simulink model "commhdlQPSKTxRxLoopback"  (R2025b)
settings: Solver=FixedStepDiscrete  StartTime=0.0  StopTime=stopTime  RelTol=1e-3
PostLoadFcn:
  | hScopeConfig = get_param([gcs '/Receiver/QPSK Rx/Frequency and Time Synchronizer/Symbol Synchronizer/No HDL/QPSK Receiver Eye Diagram'],'ScopeConfiguration');
  | 
  | hScopeConfig.OpenAtSimulationStart = false;
  | hScopeConfig.Visible = false;
  | SamplesPerSymbol = 4;
  | %UpsamplesRx = 1;
  | clear hScopeConfig
InitFcn:
  | commhdlQPSKTxRxModelInit;
  | % Rate bridge: ADRV9002/Jupiter radio runs at 15.36 MHz = 2x the 7.68 MHz
  | % (4 samples/symbol @ Rsym=1.92 MHz) the QPSK Rx requires. The deployed
  | % Receiver must downsample the ADC stream by 2. UpsamplesRx=1 fed the QPSK
  | % Rx 8 sps (2x-upsampled) and broke symbol sync / the loopback bit check.
  | UpsamplesRx = 1;   %% T8 RATE FIX: rail 15.36e6 == ADC bus rate,
  | %% no ingress decimation (was 2 when the rail sat on the 7.68e6 rung)
  | UpsamplesTx = 1;
  | clear simTimingOffset;
StopFcn:
  | if exist('simTimingOffset','var')
  |   disp('Simulation completed');
  |   %QPSKTxRxVerification;
  | end
undefined symbols (not defined in the file or in its folder): Add, Config, fsym, randsrc, RandStream, Rsym, Shift
libraries: hdlsllib x141, simulink x43, dspsigops x34, dsphdlfiltering2 x6, dsphdlsigops2 x4, dsphdlmathfun2 x4, commdigbbndpm3 x4, dspmlti4 x2, commchan3 x1, commrflib2 x1, commcnvcod2 x1
(part 7 of 8)

== matlab function commhdlQPSKTxRxLoopback/TxRxComposite/Transmitter/Input Data/Message Generator/MATLAB Function ==
  data: enable input; reset input; out output; start output; stop output; valid output; count_out output; msg_count_out output
function [out, start, stop, valid, count_out, msg_count_out] = msggen(enable, reset)

persistent indexCount;
persistent toggle;
persistent msgCount;
persistent msgCountAll;
persistent msgCountBitIndex;

if isempty(indexCount) || isempty(toggle) || isempty(msgCount) || isempty(msgCountBitIndex) || isempty(msgCountAll)
    indexCount = uint32(0);
    msgCount = uint32(1);
    msgCountAll = uint32(1);
    msgCountBitIndex = uint8(0);
    toggle = false;
end

%% Constants -- FIXED pre-coded K=5 packet ROM (rom_words_770_f1536.txt, 24640 bits,
%% word w = bits[32w..32w+31] MSB-first). Stored as 770 x uint32 packed words
%% (a large inline logical literal crashes the Stateflow compiler),
%% unpacked into the 24640-element msgbits logical ROM and indexed with the
%% STOCK msgbits(indexCount+1) pattern. Replaces the stock 120-bit message ROM.
%% Content: K=5 [35 23] rate-1/2 coded info(12292)+tail(4) -> 24592 bits,
%% 1537x16 block-interleaved (perm r*16+c), + 48-bit PN9 filler. The K=5 Rx
%% deint(perm c*1537+r) + Viterbi(TB=25) recovers the 120-bit BIST message.
romWords = uint32([1204774986 2628405925 554197542 497400430 3820996551 1221748015 2714990298 259515120 3204786136 1111747194 4265078083 2294061781 4252484111 1721148643 1557893860 2008503539 2846627651 3001288225 3608790069 3556344180 2110069204 953332885 1538372371 3729622172 3587583480 2271786194 2977718194 1348372668 2426036822 1212264446 3479632192 3945694248 146715858 66061989 1158569579 2616330249 1320555108 3805748206 240428658 3122285248 1299730390 3039860570 771131690 2822406337 4290661082 2202099387 1549769405 2893845989 2600998515 1200035258 1094107672 1099071980 3265008536 2410273076 211921841 3201301283 3732450805 450863460 3808790566 2960537398 3321481865 2122952525 1387176159 1143071442 2099631177 2056641042 2863641865 1231021455 376307909 2197616876 2437410101 3473231534 1707820516 2804199802 4287800970 525245512 4287400560 941733719 2353727255 98958867 2441609524 1877563057 3458874722 4188353559 105620265 2074471427 1983048857 720775365 1107546864 4186768650 4288099257 1794542376 3585370352 3044414555 2973237059 438542858 663684233 4210999825 3687383987 2255322999 126746480 3874147988 3557246437 2327814052 2259727769 529243390 3139808402 1019349601 2913468750 3776145438 3218192218 1679393486 3688748042 901720909 839412932 92549236 4143869516 1934824460 1788212287 1942769059 1013575849 4110032482 563053040 1850769809 3240488323 2714138779 3171475398 2388251191 1287499602 2021425911 1663633101 2002380262 1487753104 2246178129 1703254886 492327426 2325492332 2800490288 3855795855 2775932910 529157251 1196838802 2389495825 2572500611 2575775365 1699514222 108536952 2750430041 4181752401 1819429509 2974747839 355458965 2012678107 2065033890 2844786194 3112234506 448673660 1484836811 2565291703 2094477854 3409179015 3327510003 3061116728 1944795825 2928127174 3552699018 2826263714 1931323920 2645996902 3881268263 725387150 4088705762 1959664038 612041663 3911000564 2257654739 3351079667 3084688792 3456682010 1882276373 3687344633 284287204 1736971757 3103109075 4280140713 2034865353 418309356 3396932588 1653019787 2489749539 3630574176 4241866407 260297666 2207592771 1611613421 2911869622 3858688321 2102485348 2606470610 1176244465 1972735515 1070738434 351822450 561779589 3717736920 1859230250 4190007144 3344666225 3718908926 1809913940 1552395775 170097309 3420266284 1291195965 414060454 3151636196 4181278958 69544123 1722966976 41363848 2052701966 2148240930 4210020045 1643657000 1434007316 2347774674 3570790404 2646965859 460251005 539614019 1888233478 1288955089 3958237818 1648780214 1688035146 855190402 4260566109 1992029421 3644403845 1457796463 707712161 2823206006 1846212180 1982008497 2947687159 3226916667 4197619858 4061717247 1762791550 51771752 1278696143 2864974893 770780492 3533740632 3702846591 458139812 1644550038 2378873953 131264765 424436432 3448581319 3977084430 2800008767 2727081006 1655892854 2436086872 119146047 665050641 3437208595 1599135822 2504069279 388650233 3639789145 3240350459 4054822260 2241026101 2315674586 3729684387 1673449533 4151924669 1548927388 340442120 133565182 4200412650 4014554963 2830808994 3551506689 1060106442 1252542399 3144191027 1035991056 4177333083 1741372263 3444104152 2835757074 2700282813 4011008101 425083707 644064140 3120038514 52663435 441667303 1895325662 1263931564 2569151693 4193445321 3378052811 855702763 3838759059 3308062449 1762745925 482832492 4223184315 2644262910 1282602893 3423923583 650582707 2333083778 3611966168 146704471 2253469441 2443167931 2065993115 2080912288 1573737723 3314798495 1753118653 452812869 3716937464 4067956266 3742845879 778453385 2954915383 3282312798 938302038 253881325 2795823423 2048676349 1594677050 2892897791 3727926439 3354101939 4198775546 1311370449 660520948 1353333928 154880548 2183869470 3725060759 2775971433 2575221904 2416034488 1657646592 3975407894 3052635703 1492153189 1557243130 1990465897 3308726660 439225568 85633354 4136453725 1495386754 1238548381 2298304656 2764377392 3649873585 2855253402 352344240 4094790042 969194247 4109734163 2337406488 2052196884 1091394433 803488059 1420380632 3128826663 3300317325 3947491526 301996578 2469890012 364654923 1170711462 2101109723 2136067173 274042398 806681041 2016703426 65809425 3192195138 3137859966 327888233 4194535610 3421255874 3294504871 2140344047 1986028453 3808044794 2446014534 3404471016 3822490226 104670575 1409213923 1771815875 1861397759 3161897377 600711989 2495113862 98524199 3813251024 2671722550 2817217516 3002574443 2519927130 3407407452 2312290502 407193247 4039266755 501354262 3932288117 2756321076 2418573729 2458706003 1768535580 1207610603 1938379566 1394731687 722817691 1156560878 3578824878 152882305 1969362243 1045935806 1919909200 2553299454 1691462377 384797729 342156685 4135847569 2752480027 572456332 1200746083 453259896 1173847343 2353570240 459967769 2229718858 234583034 3737354549 641363899 905708352 870591043 3816338511 4226902414 2944636663 2336637460 2639437974 4034472609 2625303238 405966835 434115564 2344572364 3290037663 892007983 1420432470 3298821096 4132420023 273983924 1532258286 953608378 830848693 338305776 248034844 246724321 2408799048 736838628 2806770526 1644065415 4176725552 2124475767 3595325100 2188919204 2600844190 1349260617 2465252426 681074018 3138380009 1254671038 2934970439 1755881642 2769505031 461276217 185413998 3689401219 1367446192 571090872 1964780208 3814307016 757034307 3302748047 762001668 3679735498 728484025 766308866 748968577 674652066 2692869255 2517922336 1176671792 439389165 275378995 2836149972 490199459 3418377363 2021597030 1122295240 3220148284 3587762966 2983976142 2996338941 1116580303 3675641017 4198486036 4137897679 685212839 2993855123 2423958832 2455239403 2542605922 3900485849 3144938974 3276808451 2606275657 1746710520 1838688044 2077093415 4219364598 4244533891 1670316944 1079359898 2000045550 1670044149 188287566 2387254478 4261053412 2934638187 169533072 186361277 1903326275 4188630055 256552686 2091365340 1887121706 2640438865 3842184106 2951323892 2513539091 2511150141 781332531 542618297 2808902628 2978110120 2333290371 4245887000 93692904 1794984085 2489138070 3630290001 1119726474 2949617493 2134020159 236835366 3830512295 2972725471 3770706533 164082753 2865844902 1963690776 547110901 68479344 2796641984 2157190697 2932488526 2565680122 199251104 2750385936 802045313 3487181851 3597940860 475550533 1731466611 617462254 1433761826 836633181 1254421314 4038005858 3758110602 1598484844 1764036035 1295413010 3612526779 3138044946 1487254459 2108728938 848239132 1884273911 806105759 2310209825 2793858610 142930553 1553760878 3765966331 1562125418 2195476893 98469432 12906494 771062714 2253495211 1508761233 1665010205 3343992922 648068057 4112097869 3902847612 1022478996 3591990475 1950414917 2290204022 3154386784 871299472 1308337656 3033065682 4037020892 901499362 293410562 2019718569 954362259 339324018 519334800 1419073632 3395549952 3113043604 1078022679 810475512 1680482793 3700335650 2071919666 3304054863 1221237577 3975557103 2288714635 1595764409 4272200962 1337052842 1448452549 1029713775 2675256063 2684707814 1138561228 3133255109 2040218036 2220298315 310391 3106542365 377013759 2931553628 3732706256 3361158608 39619392 1901289326 2461657569 391876191 4064810655 2713048210 2936763192 2804600942 2365800552 2185854409 2722164045 753728523 2696644393 3850641401 4080146876 1374584058 3196598824 3331963406 1038394409 3579841592 3165824404 1180665147 4001736500 1321078348 3862082772 1172264154 818506928 2212852913 399604020 57201615 103247012 3640764147 694436346 4272012647 316665873 82210424 3660906122 3449235625 3501281049 629142576 1125610876 426370477 1297644825 1906733320 1681235753 3340101163 3791793856 1591759449 2684862014 678672541 461395676 87629339 423207683 3845784129 529695163 756923300 1075034517 2811004745 854540833 2400148390 116007136 3496921158 749261405 3687467187 3133898680 295628066 1131078894 1959427393 885629835 1375667949 3684017968 1031834568 2286756503 2220869458 312242760 2857537372 99505339 1055291367 2596856259 1592613546 2990718201 1937257331 2787897945 4159425166 2898109988 1035418457 3161449681 1840239700 1902395198 433815854 594493721 2222399192 4293104410 1184159980 2612470674 2702705650 2972371074 1574626069 3945937279 1167261571 3742839305]);
msgbits = false(1,24640);
for w = 0:769
    wv = romWords(w+1);
    for bb = 0:31
        msgbits(w*32 + bb + 1) = bitget(wv, 32 - bb) ~= uint32(0);
    end
end
msgbitsLen = uint32(length(msgbits));

fullMessageLen = uint32(24640-1); %% Need the -1 to eat the feedback delay (stock hardcoded value in this model)

%% Logic
if enable && ~reset
    %% Set out data
    if indexCount < msgbitsLen %% Emit the fixed pre-coded packet bit (unpacked ROM)
        out = msgbits(indexCount + 1);
        msgCountBitIndex = uint8(0);
    else %% beyond the ROM (should not occur: msgbitsLen==dataBitsPerPacket)
        out = false;
        msgCountBitIndex = uint8(0);
    end

    %% Flags
    start = indexCount == uint32(0);
    stop = indexCount == fullMessageLen;
    valid = true;

    %% Counters
    if fullMessageLen == indexCount
        if msgCount >= 9
            msgCount = uint32(1);
        else
            msgCount = msgCount +  1;
            msgCountAll = msgCountAll + 1;
        end
    end
    if indexCount <= fullMessageLen
        indexCount = indexCount + 1;
    end

else %% Enable == false

    if reset
        indexCount = uint32(0);
        msgCountBitIndex = uint8(0);
        toggle = false;
    end
    out = false;
    start = false;
    stop = false;
    valid = false;
end

if isempty(indexCount)
    count_out = uint32(0);
else
    count_out = indexCount;
end

msg_count_out = msgCountAll;

== matlab function commhdlQPSKTxRxLoopback/Receiver/QPSK Rx/Frequency and Time Synchronizer/Preamble Detector/FIFO/Validate Input Push Pop/MATLAB Function ==
  data: rst input; count output; enb input; dir input; initVal parameter; countToVal parameter
function count = hdlCounter(rst,enb,dir,initVal,countToVal)
%#codegen

persistent countReg

if(isempty(countReg))
    countReg = fi(initVal,0,nextpow2(countToVal+1),0);
end

if(rst)
    countReg(:) = initVal;
elseif(enb)
    if(dir)
        if(countReg==countToVal)
            countReg(:) = initVal;
        else
            countReg(:) = countReg+1;
        end
    else
        if(countReg==initVal)
            countReg(:) = countToVal;
        else
            countReg(:) = countReg-1;
        end
    end
end

count = countReg;

end

== matlab function commhdlQPSKTxRxLoopback/Receiver/QPSK Rx/Frequency and Time Synchronizer/Preamble Detector/FIFO/Validate Input Push Pop/No HDL/MATLAB Function ==
  data: pushFullDiag input; popEmptyDiag input; pushFull input; popEmpty input
function pushPopDiagnostics(pushFullDiag, popEmptyDiag, pushFull, popEmpty)
%#codegen


if(pushFull)
    switch pushFullDiag
        case 2
            warning('Push signal applied on full FIFO');
        case 3
            error('Push signal applied on full FIFO');
        otherwise
    end
end

if(popEmpty)
    switch popEmptyDiag
        case 2
            warning('Pop signal applied on empty FIFO');
        case 3
            error('Pop signal applied on empty FIFO');
        otherwise
    end
end

end

== matlab function commhdlQPSKTxRxLoopback/TxRxComposite/Transmitter/QPSK Tx/Bit Packetizer/Data Bits FIFO/MATLAB Function1 ==
  data: wr input; full output; rd input; dataBitsPerPacket parameter
function full = fcn(wr,rd,dataBitsPerPacket)
%#codegen
     
    depth = dataBitsPerPacket*2 - 1;
    persistent count;
    if isempty(count)
        count = fi(0,0,nextpow2(depth),0,hdlfimath);
    end

    if wr
        count(:) = count + 1;
    end
    if rd
        count(:) = count - 1;
    end

    full = (count > depth);

end

== matlab function commhdlQPSKTxRxLoopback/Transmitter/QPSK Tx/Bit Packetizer/Data Bits FIFO/No HDL/MATLAB Function ==
  data: wr input; full output; rd input; ncount output; empty output; dataBitsPerPacket parameter
function [full,ncount,empty] = fcn(wr,rd,dataBitsPerPacket)
%#codegen
     
    depth = dataBitsPerPacket*2 - 1;
    persistent count;
    if isempty(count)
        count = fi(0,0,nextpow2(depth),0,hdlfimath);
    end

    empty = (count == 0);
    full = (count > depth);
    ncount = count;

    if wr
        count(:) = count + 1;
    end
    if rd
        count(:) = count - 1;
    end

end

== matlab function commhdlQPSKTxRxLoopback/TxRxComposite/Transmitter/QPSK Tx/Bit Packetizer/Data Bits FIFO/No HDL/MATLAB Function ==
  data: wr input; full output; rd input; ncount output; empty output; dataBitsPerPacket parameter
function [full,ncount,empty] = fcn(wr,rd,dataBitsPerPacket)
%#codegen
     
    depth = dataBitsPerPacket*2 - 1;
    persistent count;
    if isempty(count)
        count = fi(0,0,nextpow2(depth),0,hdlfimath);
    end

    empty = (count == 0);
    full = (count > depth);
    ncount = count;

    if wr
        count(:) = count + 1;
    end
    if rd
        count(:) = count - 1;
    end

end

== matlab function commhdlQPSKTxRxLoopback/TxRxComposite/Transmitter/QPSK Tx/Bit Packetizer/Data Bits FIFO/RAM Frame Status Indicator ==
  data: push input; out output; pop input; dataBitsPerPacket parameter
function out = fcn(push,pop,dataBitsPerPacket)

   persistent pushCount popCount frameCount;
   if isempty(pushCount)
       pushCount = fi(0,0,nextpow2(dataBitsPerPacket),0,hdlfimath);
       frameCount = fi(0,0,2,0,hdlfimath);
       popCount = fi(0,0,nextpow2(dataBitsPerPacket),0,hdlfimath);
   end
   
   if (pushCount == dataBitsPerPacket-1) && push
       frameCount(:) = frameCount + 1;
   end
   if (popCount == dataBitsPerPacket-1) && pop
       frameCount(:) = frameCount - 1;
   end

   if push
       if pushCount == dataBitsPerPacket - 1
           pushCount(:) = 0;
       else
           pushCount(:) = pushCount + 1;
       end
   end

   if pop 
       if popCount == dataBitsPerPacket - 1
           popCount(:) = 0;
       else
           popCount(:) = popCount + 1;
       end
   end

   out = frameCount;

end

== matlab function commhdlQPSKTxRxLoopback/TxRxComposite/Receiver/Capture Data Bits/MATLAB Function ==
  data: valid input; datain input; start input; stop input; count_out output; packets_out output; bit_errors_out output
function [count_out, packets_out, bit_errors_out] = msgdec(valid, datain, start, stop)

persistent count;
persistent msgbuffer;

persistent packetsReceived
persistent errors;

if isempty(count) || isempty(msgbuffer) || isempty(packetsReceived)
    count = uint32(0);
    msgbuffer = zeros(1,120+8)>0; % ADI Hello WorldX
    packetsReceived = uint32(0);
    errors = uint32(0);
end

% Mesg
strAscii = dec2bin('ADI Hello World',8);
msgarray = reshape(strAscii', [1, numel(strAscii)]);
msgbits = logical(msgarray - 48);

% msgLen = uint32(2240);

if valid
    if start
        count = uint32(1);
        packetsReceived = packetsReceived + 1;
    end

    if count <= (length(msgbuffer) - 8)
        msgbuffer(count) = datain;
        if datain ~= msgbits(count)
            errors = errors + 1;
        end

    elseif count == length(msgbuffer) + 1
        msgarray_dec = char('0' + msgbuffer);
        N = length(msgarray_dec) / 8;
        strAscii_dec = reshape(msgarray_dec , 8, N).';
        msg = char(bin2dec(strAscii_dec).');
        disp(msg);
    end
    
    if count <= length(msgbuffer) + 2
        count = count + 1;
    end
end

count_out = count;
packets_out = packetsReceived;
bit_errors_out = errors;

== matlab function commhdlQPSKTxRxLoopback/TxRxComposite/Receiver/QPSK Rx/Frequency and Time Synchronizer/Packet Controller/MATLAB Function ==
  data: valid input; syncPulse input; out output
function out = fcn(valid,syncPulse)
%#codegen

  persistent Reg;
  if isempty(Reg)
      Reg = false;
  end
  
  out = Reg;
  
  if Reg && valid
      Reg = false;
  end
  
  if syncPulse
      Reg = true;
  end
  
end

== matlab function commhdlQPSKTxRxLoopback/TxRxComposite/Receiver/QPSK Rx/Frequency and Time Synchronizer/Packet Controller/sample discard controller ==
  data: dataIn input; validIn input; dataOut output; startIn input; endIn input; startOut output; endOut output; validOut output
function [dataOut,startOut,endOut,validOut] = controller(dataIn,validIn,startIn,endIn)
%#codegen

   persistent active dataOutReg validOutReg startOutReg endOutReg;
   if isempty(active)
      active  = false;
      dataOutReg = cast(0,'like',dataIn);
      validOutReg = false;
      startOutReg = false;
      endOutReg = false;
   end
   
   dataOut = dataOutReg;
   validOut = validOutReg;
   startOut = startOutReg;
   endOut = endOutReg;
   
   startOutReg = startIn;
   endOutReg = endIn;
   
   if startIn
       active = true;
   end
   
   if active
       dataOutReg(:) = dataIn;
       validOutReg = validIn;
   else
       dataOutReg(:) = 0;
       validOutReg = false;
   end
   
   if endIn
       if active 
           endOutReg = true;
       else
           endOutReg = false;
       end
       active = false;
   end
end

== matlab function commhdlQPSKTxRxLoopback/TxRxComposite/Receiver/QPSK Rx/Frequency and Time Synchronizer/Preamble Detector/Correlator/ThresholdLimiter ==
  settings: fimath=hdlfimath
  data: x input; y output
function y = applyLowerLimit(x)
    % Apply a lower limit to the threshold.
    %#codegen
    
    % Threshold is computed by summing across 63 samples.
    % Set lower limit to be equivalent of all 63 samples
    % having their LSB set to 1 and all others set to 0. 
    lowerLimit = cast(0.01, 'like', x);
    
    if x < lowerLimit
        y = lowerLimit;
    else
        y = x;
    end
end

== matlab function commhdlQPSKTxRxLoopback/TxRxComposite/Receiver/QPSK Rx/Frequency and Time Synchronizer/Preamble Detector/FIFO/Validate Input Push Pop/MATLAB Function ==
  data: rst input; count output; enb input; dir input; initVal parameter; countToVal parameter
function count = hdlCounter(rst,enb,dir,initVal,countToVal)
%#codegen

persistent countReg

if(isempty(countReg))
    countReg = fi(initVal,0,nextpow2(countToVal+1),0);
end

if(rst)
    countReg(:) = initVal;
elseif(enb)
    if(dir)
        if(countReg==countToVal)
            countReg(:) = initVal;
        else
            countReg(:) = countReg+1;
        end
    else
        if(countReg==initVal)
            countReg(:) = countToVal;
        else
            countReg(:) = countReg-1;
        end
    end
end

count = countReg;

end

== matlab function commhdlQPSKTxRxLoopback/TxRxComposite/Receiver/QPSK Rx/Frequency and Time Synchronizer/Preamble Detector/FIFO/Validate Input Push Pop/No HDL/MATLAB Function ==
  data: pushFullDiag input; popEmptyDiag input; pushFull input; popEmpty input
function pushPopDiagnostics(pushFullDiag, popEmptyDiag, pushFull, popEmpty)
%#codegen


if(pushFull)
    switch pushFullDiag
        case 2
            warning('Push signal applied on full FIFO');
        case 3
            error('Push signal applied on full FIFO');
        otherwise
    end
end

if(popEmpty)
    switch popEmptyDiag
        case 2
            warning('Pop signal applied on empty FIFO');
        case 3
            error('Pop signal applied on empty FIFO');
        otherwise
    end
end

end

== matlab function commhdlQPSKTxRxLoopback/Receiver/QPSK Rx/Frequency and Time Synchronizer/Packet Controller/MATLAB Function ==
  data: valid input; syncPulse input; out output
function out = fcn(valid,syncPulse)
%#codegen

  persistent Reg;
  if isempty(Reg)
      Reg = false;
  end
  
  out = Reg;
  
  if Reg && valid
      Reg = false;
  end
  
  if syncPulse
      Reg = true;
  end
  
end

== matlab function commhdlQPSKTxRxLoopback/TxRxComposite/Receiver/QPSK Rx/Frequency and Time Synchronizer/Symbol Synchronizer/Interpolation Control ==
  data: mu output; Delta input; Underflow output
function [mu,Underflow] = Interpolation_ctrl(Delta)
% Implementation of modulo-1 counter for interpolation control listed in
% Figure 8.4.19 of "Digital Communications - A Discrete-Time Approach"
% by Michael Rice. See design details in Chapter 8.4.3 of the same book.
% 
% Input:
%   Delta - Loop filter output. If loop is in lock, delta would be small
% Output:
%   Underflow - Indicator of counter underflow. This is the strobe signal
%               for downstream processing
%   mu - Difference between actual sampling instant and the optimal instant,
%        between zero and one
%#codegen

% countReg - Counter value delayed by 1 sample
% muReg - The estimated timing error normalized by half QPSK symbols

   mask = fi(1-2^(-10),1,11,10);
   
   persistent countReg underflowReg muReg;
   if isempty(countReg)
       countReg  = fi(0,1,11,10);
       muReg = fi(0,1,11,10);
       underflowReg = false;
   end
   
   
   Underflow = underflowReg;
   mu = muReg;   
   
   
      % T8.4 anti-wedge clamp: if Delta <= -0.125 the decrementing counter
   % never underflows (strobes stop FOREVER -- Class-4 wedge / Class-1
   % episode mechanism; see tb_timing_wedge.v). Bound Delta so the
   % counter always decrements by >= 1 LSB.
   wlim = fi(255/1024,1,11,10);
   if Delta > wlim
       Delta = wlim;
   elseif Delta < -wlim
       Delta = fi(-255/1024,1,11,10);
   end
   counter = bitand(mask,countReg)-Delta-fi(0.25,1,11,10); % decrementing counter
   
   % if countReg is a nonnegative number,
   % then mod(countReg,1) equals the fractional part of countReg
   if counter < 0
       underflowReg = true;
       muReg = bitshift(bitand(mask,countReg),2);
       countReg = fi(counter+1,1,11,10);% create underflow to counter
   else
       underflowReg = false;
       countReg = fi(counter,1,11,10);
   end
   


end

== matlab function commhdlQPSKTxRxLoopback/TxRxComposite/Receiver/QPSK Rx/Frequency and Time Synchronizer/Symbol Synchronizer/Rate Handle/FIFO/Validate Input Push Pop/MATLAB Function ==
  data: rst input; count output; enb input; dir input; initVal parameter; countToVal parameter
function count = hdlCounter(rst,enb,dir,initVal,countToVal)
%#codegen

persistent countReg

if(isempty(countReg))
    countReg = fi(initVal,0,nextpow2(countToVal+1),0);
end

if(rst)
    countReg(:) = initVal;
elseif(enb)
    if(dir)
        if(countReg==countToVal)
            countReg(:) = initVal;
        else
            countReg(:) = countReg+1;
        end
    else
        if(countReg==initVal)
            countReg(:) = countToVal;
        else
            countReg(:) = countReg-1;
        end
    end
end

count = countReg;

end

== matlab function commhdlQPSKTxRxLoopback/TxRxComposite/Receiver/QPSK Rx/Frequency and Time Synchronizer/Symbol Synchronizer/Rate Handle/FIFO/Validate Input Push Pop/No HDL/MATLAB Function ==
  data: pushFullDiag input; popEmptyDiag input; pushFull input; popEmpty input
function pushPopDiagnostics(pushFullDiag, popEmptyDiag, pushFull, popEmpty)
%#codegen


if(pushFull)
    switch pushFullDiag
        case 2
            warning('Push signal applied on full FIFO');
        case 3
            error('Push signal applied on full FIFO');
        otherwise
    end
end

if(popEmpty)
    switch popEmptyDiag
        case 2
            warning('Pop signal applied on empty FIFO');
        case 3
            error('Pop signal applied on empty FIFO');
        otherwise
    end
end

end

== matlab function commhdlQPSKTxRxLoopback/TxRxComposite/Receiver/QPSK Rx/FEC Decoder Wrapper/RxDeint ==
  data: dataIn input; codedPair output; startIn input; endIn input; validIn input; vitReset output; deintValid output; frameStart output; frameEnd output
function [codedPair, vitReset, deintValid, frameStart, frameEnd] = fecRxDeint(dataIn, startIn, endIn, validIn)
%#codegen
persistent ramA ramB rdBank wptr pcnt hold0 hold1 rdGate rcol rrow;
CODED=uint16(24592); COLS=uint16(16); ROWS=uint16(1537);
NPAIR=uint16(12296);
if isempty(ramA), ramA=fi(zeros(1,24592),0,1,0); ramB=fi(zeros(1,24592),0,1,0); rdBank=false; wptr=uint16(0); pcnt=uint16(0); hold0=fi(0,0,1,0); hold1=fi(0,0,1,0); rdGate=false; rcol=uint16(0); rrow=uint16(0); end
rb=rdBank; w=wptr; pc=pcnt; g=rdGate; h0=hold0; h1=hold1; cc=rcol; rr=rrow;
pair0=h0; pair1=h1;
vitReset=false; deintValid=false; frameStart=false; frameEnd=false;
wrPos=uint16(65535); wrBit=fi(0,0,1,0); wrBankA=false; doWr=false;
if validIn
  if startIn, w=uint16(0); pc=uint16(0); rb=~rb; g=true; cc=uint16(0); rr=uint16(0); end % rdGate=TRUE: frame pair0 read COINCIDES with frameStart (RxAlign arms on that beat); read-counters reset in lockstep with pc
  % ---- READ side first (opposite bank; RXROOT E8 isolated reads: 1 pair per 2 validIn beats) ----
  if g && (pc < NPAIR)
    % divisionless read address: cc (even col) / rr (row) are incremental counters.
    % rc0=2*pc is even so rc1=rc0+1 keeps the same row -> perm1 = perm0 + ROWS (one add).
    perm0 = cc*ROWS + rr;
    perm1 = perm0 + ROWS;
    b0v = fi(0,0,1,0); b1v = fi(0,0,1,0);
    if perm0 < CODED
      if rb, b0v = ramB(double(perm0)+1); else b0v = ramA(double(perm0)+1); end
    end
    if perm1 < CODED
      if rb, b1v = ramB(double(perm1)+1); else b1v = ramA(double(perm1)+1); end
    end
    pair0 = b0v; pair1 = b1v; h0 = b0v; h1 = b1v;
    deintValid = true;
    if pc == uint16(0), vitReset = true; end
    pc = pc + 1;
    cc = cc + uint16(2);
    if cc == COLS, cc = uint16(0); rr = rr + uint16(1); end
  end
  % ---- WRITE side after all reads ----
  if w < CODED
    wrPos = w; wrBit = fi(dataIn,0,1,0); wrBankA = rb; doWr = true;
    w = w + 1;
  end
  g = ~g;
  frameStart=startIn; frameEnd=endIn;
end
codedPair = fi([pair0; pair1], 0, 1, 0);
% ---- persist state last ----
if doWr
  if wrBankA, ramA(double(wrPos)+1)=wrBit; else ramB(double(wrPos)+1)=wrBit; end
end
rdBank=rb; wptr=w; pcnt=pc; rdGate=g; hold0=h0; hold1=h1; rcol=cc; rrow=rr;

== matlab function commhdlQPSKTxRxLoopback/TxRxComposite/Receiver/QPSK Rx/FEC Decoder Wrapper/RxAlign ==
  data: decBit input; dataOut output; deintValid input; frameStart input; frameEnd input; skipCount input; startOut output; endOut output; validOut output
function [dataOut, startOut, endOut, validOut] = fecRxAlign(decBit, deintValid, frameStart, frameEnd, skipCount)
%#codegen
persistent oc started skip;
INFO=uint16(12292);
if isempty(oc), oc=uint16(0); started=false; skip=uint16(0); end
o=oc; st=started; sk=skip;
dataOut=false; startOut=false; endOut=false; validOut=false;
sc = uint16(skipCount);
if sc > INFO, sc = INFO; end
if deintValid
  if frameStart, o=uint16(0); st=true; sk=sc+uint16(41); end % +41 = gated-Viterbi latency in deintValid beats incl. VitGate hold reg (RXROOT E8)
  if st
    if sk > uint16(0)
      sk = sk - uint16(1);
    elseif o < INFO
      dataOut = decBit;
      startOut = (o==uint16(0));
      endOut   = (o==(INFO-1));
      validOut = true;
      o = o + uint16(1);
    end
  end
end
oc=o; started=st; skip=sk;

== matlab function commhdlQPSKTxRxLoopback/TxRxComposite/Receiver/QPSK Rx/FEC Decoder Wrapper/FecCounters ==
  data: e1 input; c1 output; e2 input; e3 input; e4 input; e5 input; e6 input; c2 output; c3 output; c4 output; c5 output; c6 output
function [c1, c2, c3, c4, c5, c6] = fecCounters(e1, e2, e3, e4, e5, e6)
%#codegen
% Free-running FEC-Rx datapath event counters (reset by modem soft-reset 0x000).
persistent k1 k2 k3 k4 k5 k6;
if isempty(k1)
  k1=uint32(0); k2=uint32(0); k3=uint32(0); k4=uint32(0); k5=uint32(0); k6=uint32(0);
end
MAX=uint32(4294967295);
n1=k1; n2=k2; n3=k3; n4=k4; n5=k5; n6=k6;
if e1 && n1<MAX, n1=n1+uint32(1); end
if e2 && n2<MAX, n2=n2+uint32(1); end
if e3 && n3<MAX, n3=n3+uint32(1); end
if e4 && n4<MAX, n4=n4+uint32(1); end
if e5 && n5<MAX, n5=n5+uint32(1); end
if e6 && n6<MAX, n6=n6+uint32(1); end
c1=n1; c2=n2; c3=n3; c4=n4; c5=n5; c6=n6;
k1=n1; k2=n2; k3=n3; k4=n4; k5=n5; k6=n6;

== matlab function commhdlQPSKTxRxLoopback/Receiver/QPSK Rx/Frequency and Time Synchronizer/Symbol Synchronizer/Rate Handle/FIFO/Validate Input Push Pop/MATLAB Function ==
  data: rst input; count output; enb input; dir input; initVal parameter; countToVal parameter
function count = hdlCounter(rst,enb,dir,initVal,countToVal)
%#codegen

persistent countReg

if(isempty(countReg))
    countReg = fi(initVal,0,nextpow2(countToVal+1),0);
end

if(rst)
    countReg(:) = initVal;
elseif(enb)
    if(dir)
        if(countReg==countToVal)
            countReg(:) = initVal;
        else
            countReg(:) = countReg+1;
        end
    else
        if(countReg==initVal)
            countReg(:) = countToVal;
        else
            countReg(:) = countReg-1;
        end
    end
end

count = countReg;

end

== matlab function commhdlQPSKTxRxLoopback/TxRxComposite/Receiver/QPSK Rx/FEC Decoder Wrapper/FecCapture ==
  data: bitsIn input; capIn output; validIn input; startIn input; codedPair input; deintValid input; decBit input; skipCount input; outValid input; capDeint output; capOut output
function [capIn, capDeint, capOut] = fecCapture(bitsIn, validIn, startIn, codedPair, deintValid, decBit, skipCount, outValid)
%#codegen
persistent rIn rDe rOu nIn nDe nOu armIn skp;
if isempty(rIn)
  rIn=uint32(0); rDe=uint32(0); rOu=uint32(0);
  nIn=uint16(0); nDe=uint16(0); nOu=uint16(0); armIn=false; skp=uint16(0);
end
% sync-semantics compliant (RXROOT E11c): locals, persist last.
a=rIn; b=rDe; c=rOu; xIn=nIn; xDe=nDe; xOu=nOu; arm=armIn; sk=skp; %#ok<NASGU>
% --- CAP_IN: first 32 coded-in bits, armed at startIn, gated by validIn ---
if validIn
  if startIn, xIn=uint16(0); a=uint32(0); arm=true; end
  if arm && xIn < uint16(32)
    if bitsIn, a = bitor(a, bitshift(uint32(1), double(xIn))); end
    xIn = xIn + uint16(1);
  end
end
% --- CAP_DEINT: first 32 deint-output coded bits (2 per pair), gated by deintValid ---
if startIn, xDe=uint16(0); b=uint32(0); end
if deintValid && xDe < uint16(32)
  b0 = codedPair(1) ~= 0; b1 = codedPair(2) ~= 0;
  if b0, b = bitor(b, bitshift(uint32(1), double(xDe))); end
  xDe = xDe + uint16(1);
  if xDe < uint16(32)
    if b1, b = bitor(b, bitshift(uint32(1), double(xDe))); end
    xDe = xDe + uint16(1);
  end
end
% --- CAP_OUT (RXROOT E8): first 32 bits of the WRAPPER OUTPUT stream ---
% i6 = RxAlign dataOut gated by i8 = RxAlign validOut: exactly the bits the
% BIST compares, alignment-independent. Golden expectation 0x04922282.
sc = uint16(skipCount); sk = uint16(0); %#ok<NASGU>
if startIn, xOu=uint16(0); c=uint32(0); end
if outValid && xOu < uint16(32)
  if decBit, c = bitor(c, bitshift(uint32(1), double(xOu))); end
  xOu = xOu + uint16(1);
end
capIn = a; capDeint = b; capOut = c;
rIn=a; rDe=b; rOu=c; nIn=xIn; nDe=xDe; nOu=xOu; armIn=arm; skp=sk;

== matlab function commhdlQPSKTxRxLoopback/TxRxComposite/Receiver/QPSK Rx/FecCaptureCadence ==
  data: startIn input; capCad output; validIn input
function capCad = fecCaptureCadence(startIn, validIn)
%#codegen
persistent sCnt gap snv vrun seenStart sawValid measuring;
if isempty(sCnt)
  sCnt=uint8(0); gap=uint8(0); snv=uint8(0); vrun=uint8(0);
  seenStart=false; sawValid=false; measuring=false;
end
% sync-semantics compliant (RXROOT E11c): locals, persist last.
sC=sCnt; gp=gap; sv=snv; vr=vrun; seen=seenStart; saw=sawValid; mea=measuring;
if startIn
  if sC < uint8(255), sC = sC + uint8(1); end
  if ~validIn && sv < uint8(255), sv = sv + uint8(1); end
  if ~seen
    seen = true; mea = true; gp = uint8(0); saw=false; vr=uint8(0);
  end
end
if mea && ~saw
  if validIn
    saw = true;
  elseif gp < uint8(255)
    gp = gp + uint8(1);
  end
end
if seen && validIn && vr < uint8(255)
  vr = vr + uint8(1);
end
capCad = bitor(bitor(uint32(sC), bitshift(uint32(gp),8)), bitor(bitshift(uint32(sv),16), bitshift(uint32(vr),24)));
sCnt=sC; gap=gp; snv=sv; vrun=vr; seenStart=seen; sawValid=saw; measuring=mea;

== matlab function commhdlQPSKTxRxLoopback/TxRxComposite/Receiver/QPSK Rx/RstCsCounter ==
  data: e input; c output
function c = rstCsCount(e)
%#codegen
% Count RISING EDGES of the CFO-step-detector carrier-sync reset (AXI 0x150).
% Saturating; reset by the modem soft-reset 0x000 via the persistent init.
persistent prev cnt;
if isempty(prev), prev = false; cnt = uint32(0); end
n = cnt;
if e && ~prev && n < uint32(4294967295)
    n = n + uint32(1);
end
c = n;
cnt = n;
prev = logical(e);

== matlab function commhdlQPSKTxRxLoopback/TxRxComposite/Transmitter/Input Data/ByteBitShifter ==
  data: enable input; bit output; reset input; start input; extWord input; extWordAvail input; extWordFirst input; popToggle output
function [bit, popToggle] = byteBitShifterBlk(enable, reset, start, extWord, extWordAvail, extWordFirst)
% Block wrapper around qpskByteBitShifterStrict (the unit-tested single source
% of truth). Persistent state only; the effective enable matches the
% Message Generator chart's active condition (enable && ~reset) so the
% shifter emits bits on exactly the generator's bit steps. pop is
% exported as a toggle (one flip per word latch OR discard) to survive
% the slow->fast rate crossing; upstream edge-detects it into a pulse.
persistent state tog
if isempty(state)
    state = qpskByteBitShifterStrict();
    tog = false;
end
en = logical(enable) && ~logical(reset);
[bit, pop, state] = qpskByteBitShifterStrict(state, en, logical(start), ...
    uint64(extWord), logical(extWordAvail), logical(extWordFirst));
if pop
    tog = ~tog;
end
popToggle = tog;

== matlab function commhdlQPSKTxRxLoopback/TxRxComposite/Transmitter/Input Data/FEC Tx Encoder K5/TxGateK5 ==
  data: bitIn input; infoBit output; enable input; reset input; start input; encReset output; infoValid output; beatIdx output; frameValid output; frameStart output
function [infoBit, encReset, infoValid, beatIdx, frameValid, frameStart] = fecTxGateK5(bitIn, enable, reset, start)
%#codegen
% sync-semantics (RXROOT E11c): locals in, outputs from locals, persist last.
persistent beat armed;
INFO=uint16(12292); NIN=uint16(12296); PAYLOAD=uint16(24640);
if isempty(beat), beat=uint16(0); armed=false; end
b=beat; a=armed;
infoBit=false; encReset=false; infoValid=false; beatIdx=uint16(0);
frameValid=false; frameStart=false;
en = logical(enable) && ~logical(reset);
if en
  if start, b=uint16(0); a=true; encReset=true; end
  if a
    if b < INFO
      infoBit = logical(bitIn); infoValid = true;
    elseif b < NIN
      infoBit = false;          infoValid = true;   % K-1 zero tail flush
    end
    beatIdx = b; frameValid = true; frameStart = (b==uint16(0));
    if b < PAYLOAD-uint16(1), b=b+uint16(1); else, b=uint16(0); end
  end
end
beat=b; armed=a;

== matlab function commhdlQPSKTxRxLoopback/TxRxComposite/Transmitter/Input Data/FEC Tx Encoder K5/ConvEncK5 ==
  data: infoBit input; codedPair output; encReset input; infoValid input
function codedPair = fecConvEncK5(infoBit, encReset, infoValid)
%#codegen
persistent sr;
if isempty(sr), sr = false(1,4); end
srUse = sr;
if encReset, srUse = false(1,4); end   % reset-then-advance (zero frame state)
in = logical(infoBit);
s0=in; s1=srUse(1); s2=srUse(2); s3=srUse(3); s4=srUse(4);
g0 = xor(s0, xor(s1, xor(s2, s4)));   % poly 35 oct = 11101
g1 = xor(s0, xor(s3, s4));            % poly 23 oct = 10011
codedPair = [g0; g1];
% state update: advance ONLY on infoValid, else HOLD (anti-zero-stuff gate)
if infoValid
  sr = [in, srUse(1:3)];
else
  sr = srUse;
end

== matlab function commhdlQPSKTxRxLoopback/TxRxComposite/Transmitter/Input Data/FEC Tx Encoder K5/TxInterleaveK5 ==
  data: codedPair input; dataOut output; infoValid input; beatIdx input; frameValid input; frameStart input
function dataOut = fecTxInterleaveK5(codedPair, infoValid, beatIdx, frameValid, frameStart)
%#codegen
persistent ramA ramB rdBank wptr rrow rcol;
CODED=uint16(24592); COLS=uint16(16); ROWS=uint16(1537);
FILL = logical([1 1 1 1 1 1 1 1 1 0 0 0 0 0 1 1 1 1 0 1 1 1 1 1 0 0 0 1 0 1 1 1 0 0 1 1 0 0 1 0 0 0 0 0 1 0 0 1]);   % 64-bit PN9 filler (T8 fix 6bcaa62)
if isempty(ramA), ramA=fi(zeros(1,24592),0,1,0); ramB=fi(zeros(1,24592),0,1,0); rdBank=false; wptr=uint16(0); rrow=uint16(0); rcol=uint16(0); end
rb=rdBank; w=wptr; rr=rrow; cc=rcol;
dataOut=false;
wr0=uint16(0); wr1=uint16(0); v0=fi(0,0,1,0); v1=fi(0,0,1,0); doW0=false; doW1=false;
if frameValid
  if frameStart, w=uint16(0); rb=~rb; end
  % ---- READ side (previous frame, opposite bank), legacy perm r*COLS+c ----
  % divisionless read address: rr (row 0..ROWS-1) / cc (col 0..COLS-1) are
  % incremental counters, reset on beatIdx==0, advancing +1 row with col carry
  % per in-range beat -- replaces the old per-beat divide-by-ROWS. No divide.
  if beatIdx < CODED
    % precondition: bit-exactness requires a contiguous beatIdx hitting 0 once per
    % frame to re-seed the row/col counters (the old stateless per-beat address
    % arithmetic derived the address from beatIdx alone and needed no such reset).
    if beatIdx == 0, rr = uint16(0); cc = uint16(0); end
    perm = rr*COLS + cc;
    if perm < CODED
      if rb, dataOut = logical(ramB(double(perm)+1)); else, dataOut = logical(ramA(double(perm)+1)); end
    end
    rr = rr + uint16(1);
    if rr == ROWS, rr = uint16(0); cc = cc + uint16(1); end
  else
    dataOut = FILL(double(beatIdx-CODED)+1);   % PN9 filler, beats CODED..2239
  end
  % ---- WRITE side: two coded bits per encoder-advance beat ----
  if infoValid
    if w < CODED, wr0=w; v0=fi(double(codedPair(1)~=0),0,1,0); doW0=true; w=w+uint16(1); end
    if w < CODED, wr1=w; v1=fi(double(codedPair(2)~=0),0,1,0); doW1=true; w=w+uint16(1); end
  end
end
% ---- persist state last (write bank = opposite of read bank) ----
if doW0
  if rb, ramA(double(wr0)+1)=v0; else, ramB(double(wr0)+1)=v0; end
end
if doW1
  if rb, ramA(double(wr1)+1)=v1; else, ramB(double(wr1)+1)=v1; end
end
rdBank=rb; wptr=w; rrow=rr; rcol=cc;

== matlab function commhdlQPSKTxRxLoopback/TxRxComposite/ByteWordBuffer ==
  data: dataIn input; word output; validIn input; popReq input; firstIn input; avail output; readyNext output; wordFirst output
function [word, avail, readyNext, wordFirst] = byteWordBufferBlk(dataIn, validIn, popReq, firstIn)
% Block wrapper around qpskByteWordBufferSkid (unit-tested single source of
% truth); persistent state only. readyNext = the post-update registered
% ready; an external Delay (IC=1) turns it back into the AXIS tready.
% firstIn/wordFirst carry the in-band first-word marker alongside data.
persistent state
if isempty(state)
    state = qpskByteWordBufferSkid();
end
[word, avail, ~, wordFirst, state] = qpskByteWordBufferSkid(state, uint64(dataIn), ...
    logical(validIn), logical(popReq), logical(firstIn));
readyNext = state.readyReg;

== matlab function commhdlQPSKTxRxLoopback/TxRxComposite/ByteSerializer ==
  data: bitIn input; word output; bitValid input; start input; ready input; wordTog output; wordLast output; wordFirst output
function [word, wordTog, wordLast, wordFirst] = byteSerializerBlk(bitIn, bitValid, start, ready)
% Block wrapper around qpskByteSerializer (unit-tested single source of
% truth); persistent state only. word/wordLast are HELD stable between
% emissions; wordTog flips once per emitted word so the slow->fast rate
% crossing cannot drop or repeat it -- the 30.72M BeatGate edge-detects
% it into exactly one accepted AXIS beat. Dropped words (ready low at
% completion) do not toggle: drop means NO beat, never a stall.
% K5 kit: 191 words/frame = the first 64*191 of
% the 1084 decoded info bits; the trailing 60 are dropped by start-reset.
persistent state tog heldWord heldLast heldFirst firstNext
if isempty(state)
    state = qpskByteSerializer();
    tog = false; heldWord = uint64(0); heldLast = false;
    heldFirst = true; firstNext = true;
end
% presentation is decoupled from acceptance (ADI S2MM source style):
% the offered beat must refresh on EVERY completed word or the DMA's
% SYNC_TRANSFER_START gate can wait forever on a frozen user flag /
% accept a stale word. ready at the pin only decides acceptance, so
% the core serializer runs with ready=true and unaccepted beats are
% simply superseded.
[w, wv, wl, ~, state] = qpskByteSerializer(state, logical(bitIn), ...
    logical(bitValid), logical(start), true, uint16(191));
if wv
    heldWord = w; heldLast = logical(wl); tog = ~tog;
    heldFirst = firstNext; firstNext = logical(wl);
end
word = heldWord; wordTog = tog; wordLast = heldLast; wordFirst = heldFirst;

== matlab function commhdlQPSKTxRxLoopback/TxRxComposite/ByteRxFifo ==
  data: word input uint64; outWord output uint64; tog input boolean; wLast input boolean; wFirst input boolean; ready input boolean; valid output boolean; outLast output boolean; outFirst output boolean; ovf output uint32
function [outWord, valid, outLast, outFirst, ovf] = byteRxFifo(word, tog, wLast, wFirst, ready)
%#codegen
% 64-deep elastic FIFO: enqueue on serializer toggle edge, dequeue on
% accepted AXIS beat. Drop-newest + count on full (stall > ~19 ms).
% f1536 SOF-prime guard (TXMUX 2026-07-25): valid is presented only after
% ready has been continuously high for 6 cycles, so the axi_dmac S2MM
% per-descriptor SOF prime (5-cycle latency, replicates a HELD beat x5 =
% the W0x5 dup) never sees a held beat during its prime window.
persistent mem memFl wr rd prev ovfCnt rdyRun
if isempty(wr)
    mem = zeros(64,1,'uint64'); memFl = zeros(64,1,'uint8');
    wr = uint16(0); rd = uint16(0); prev = false; ovfCnt = uint32(0);
    rdyRun = uint8(0);
end
if logical(tog) ~= prev
    nxt = uint16(mod(uint32(wr) + 1, 64));
    if nxt == rd
        rd = uint16(mod(uint32(rd) + 1, 64));
        ovfCnt = ovfCnt + uint32(1);
    end
    mem(uint32(wr)+1)   = uint64(word);
    memFl(uint32(wr)+1) = uint8(wLast) + uint8(2)*uint8(wFirst);
    wr = nxt;
end
prev = logical(tog);
valid = (wr ~= rd) && (rdyRun >= uint8(6));
outWord  = mem(uint32(rd)+1);
fl = memFl(uint32(rd)+1);
outLast  = bitand(fl, uint8(1)) ~= uint8(0);
outFirst = bitand(fl, uint8(2)) ~= uint8(0);
if valid && logical(ready)
    rd = uint16(mod(uint32(rd) + 1, 64));
end
if logical(ready)
    if rdyRun < uint8(255), rdyRun = rdyRun + uint8(1); end
else
    rdyRun = uint8(0);
end
ovf = ovfCnt;

== matlab function commhdlQPSKTxRxLoopback/Transmitter/QPSK Tx/Bit Packetizer/Data Bits FIFO/MATLAB Function1 ==
  data: wr input; full output; rd input; dataBitsPerPacket parameter
function full = fcn(wr,rd,dataBitsPerPacket)
%#codegen
     
    depth = dataBitsPerPacket*2 - 1;
    persistent count;
    if isempty(count)
        count = fi(0,0,nextpow2(depth),0,hdlfimath);
    end

    if wr
        count(:) = count + 1;
    end
    if rd
        count(:) = count - 1;
    end

    full = (count > depth);

end

== matlab function commhdlQPSKTxRxLoopback/TxRxComposite/Receiver/QPSK Rx/Frequency and Time Synchronizer/Preamble Detector/PdTelemetry ==
  data: validIn input boolean; telI output fixdt(1,16,0); dI input int16; dQ input int16; thrEx input boolean; tRef input uint16; tOff input uint16; done input boolean; newPk input boolean; succ input boolean; sync input boolean; armed input boolean; taRef input uint16; accOff input uint16; fifoEnt input uint16; vPop input boolean; tRefLong input uint32; runMax input uint32; heldTs input uint32; telQ output fixdt(1,16,0)
function [telI, telQ] = pdTelemetry(validIn, dI, dQ, thrEx, tRef, tOff, done, newPk, succ, sync, armed, taRef, accOff, fifoEnt, vPop, tRefLong, runMax, heldTs)
%#codegen
persistent slot symCtr beatCnt aDone aNewPk aThrEx aSync aVPop s0 s1 s2 s3 s4 s5 s6
if isempty(slot)
    slot = uint8(7); symCtr = uint32(0); beatCnt = uint8(0);
    aDone = false; aNewPk = false; aThrEx = false; aSync = false; aVPop = false;
    s0 = uint32(0); s1 = uint32(0); s2 = uint32(0); s3 = uint32(0);
    s4 = uint32(0); s5 = uint32(0); s6 = uint32(0);
end
aDone = aDone || done; aNewPk = aNewPk || newPk; aThrEx = aThrEx || thrEx;
aSync = aSync || sync; aVPop = aVPop || vPop;
if beatCnt < uint8(7), beatCnt = beatCnt + uint8(1); end
if validIn
    symCtr = symCtr + uint32(1);
    flags = uint32(aDone) + bitshift(uint32(aNewPk),1) + bitshift(uint32(succ),2) + ...
            bitshift(uint32(aThrEx),3) + bitshift(uint32(aSync),4) + bitshift(uint32(armed),5);
    s0 = bitor(bitor(bitor(bitshift(uint32(14),28), bitshift(uint32(bitand(tRef,uint16(2047))),17)), ...
         bitshift(uint32(bitand(tOff,uint16(2047))),6)), flags);
    s1 = bitor(bitshift(uint32(reinterpretcast(dI,numerictype(0,16,0))),16), ...
         uint32(reinterpretcast(dQ,numerictype(0,16,0))));
    s2 = bitor(bitor(bitor(bitshift(uint32(bitand(taRef,uint16(2047))),21), ...
         bitshift(uint32(bitand(accOff,uint16(2047))),10)), ...
         bitshift(uint32(bitand(fifoEnt,uint16(511))),1)), uint32(aVPop));
    s3 = tRefLong;
    s4 = runMax;
    s5 = heldTs;
    s6 = bitor(bitor(bitshift(uint32(165),24), bitshift(uint32(bitand(uint16(beatCnt),uint16(7))),21)), ...
         bitand(symCtr,uint32(2097151)));
    aDone = false; aNewPk = false; aThrEx = false; aSync = false; aVPop = false;
    beatCnt = uint8(0);
    slot = uint8(0);
end
switch slot
  case uint8(0), w = s0;
  case uint8(1), w = s1;
  case uint8(2), w = s2;
  case uint8(3), w = s3;
  case uint8(4), w = s4;
  case uint8(5), w = s5;
  case uint8(6), w = s6;
  otherwise,     w = uint32(0);
end
if slot < uint8(7), slot = slot + uint8(1); end
telI = reinterpretcast(uint16(bitshift(w, -16)), numerictype(1,16,0));
telQ = reinterpretcast(uint16(bitand(w, uint32(65535))), numerictype(1,16,0));

== matlab function commhdlQPSKTxRxLoopback/TxRxComposite/Receiver/QPSK Rx/Frequency and Time Synchronizer/Carrier Synchronizer/Loop Filter/LGMux_cs_prop_gain ==
  data: axi input; coeff output; nz output
function [coeff, nz] = cs_prop_gain_mux(axi)
%#codegen
nz = axi ~= uint32(0);
si = bitsliceget(axi, 16, 1);
coeff = reinterpretcast(si, numerictype(0, 16, 16));
end

== matlab function commhdlQPSKTxRxLoopback/TxRxComposite/Receiver/QPSK Rx/Frequency and Time Synchronizer/Carrier Synchronizer/Loop Filter/LGMux_cs_integ_gain ==
  data: axi input; coeff output; nz output
function [coeff, nz] = cs_integ_gain_mux(axi)
%#codegen
nz = axi ~= uint32(0);
si = bitsliceget(axi, 16, 1);
coeff = reinterpretcast(si, numerictype(0, 16, 16));
end

== matlab function commhdlQPSKTxRxLoopback/TxRxComposite/Receiver/QPSK Rx/Frequency and Time Synchronizer/Symbol Synchronizer/Loop Filter/LGMux_ss_prop_gain ==
  data: axi input; coeff output; nz output
function [coeff, nz] = ss_prop_gain_mux(axi)
%#codegen
nz = axi ~= uint32(0);
si = bitsliceget(axi, 24, 1);
coeff = reinterpretcast(si, numerictype(1, 24, 24));
end

== matlab function commhdlQPSKTxRxLoopback/TxRxComposite/Receiver/QPSK Rx/Frequency and Time Synchronizer/Symbol Synchronizer/Loop Filter/LGMux_ss_integ_gain ==
  data: axi input; coeff output; nz output
function [coeff, nz] = ss_integ_gain_mux(axi)
%#codegen
nz = axi ~= uint32(0);
si = bitsliceget(axi, 24, 1);
coeff = reinterpretcast(si, numerictype(1, 24, 24));
end

== matlab function commhdlQPSKTxRxLoopback/TxRxComposite/Receiver/QPSK Rx/Automatic Gain Control/Loop Filter/LGMux_agc_loop_gain ==
  data: axi input; coeff output; nz output
function [coeff, nz] = agc_loop_gain_mux(axi)
%#codegen
nz = axi ~= uint32(0);
si = bitsliceget(axi, 32, 1);
coeff = reinterpretcast(si, numerictype(0, 32, 31));
end
